simulink model "GaN_Full_Bridge_SPS"  (R2022b)
settings: Solver=ode45  StartTime=0.0  StopTime=55e-6  MaxStep=5e-9  RelTol=1e-7  AbsTol=1e-8
model workspace (MAT data in the model file):
  p.VDC = 150
  p.L = 9e-05
  p.Cdc = 0.0005
  p.Ron = 0.08
  p.Rdut = 0.08
  p.Raux = 0.08
  p.Rshunt = 0.01
  p.Rload = 0.001
  p.T0 = 2e-06
  p.Tcharge = 3.25e-05
  p.Tfree = 1e-06
  p.Tmeasure = 5e-06
  p.direction = 1
  p.conventional = 0
  p.idleUpper = 1
values from neighbouring files (symbols this model uses):
  p = h.(side)(index);end    [build_and_run_simulink.m]    (also in run_bridge_snapshot.m = evalin(w,'p'))
libraries: spsIdealSwitchLib x5, spsSeriesRLCBranchLib x3, spsVoltageMeasurementLib x2, spsCurrentMeasurementLib x2, spsGroundLib x1, sps_lib x1
settings Model: Creator=Greatlovers  LastModifiedBy=Greatlovers

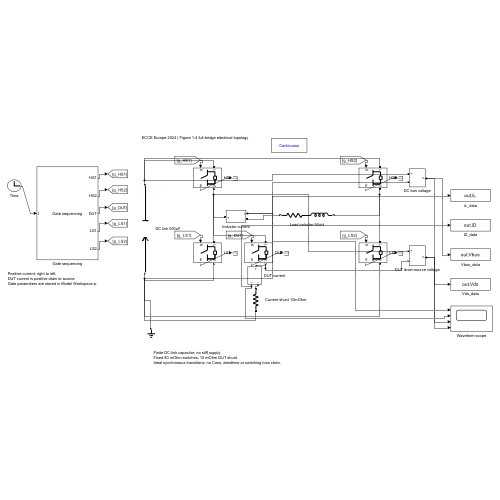
[thumbnail: Simulink's stored preview of the top-level diagram]
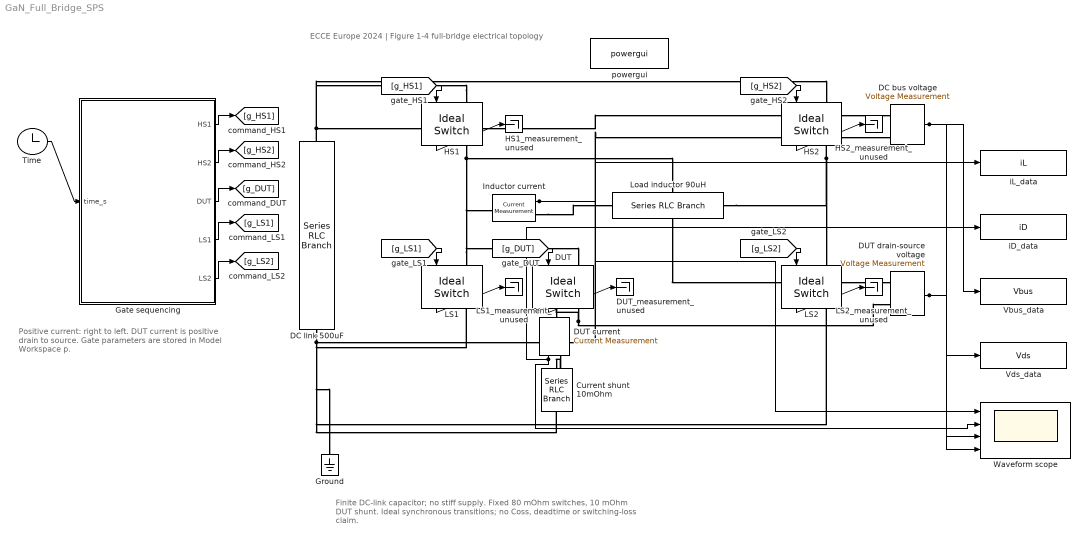
== system GaN_Full_Bridge_SPS ==
  note: ECCE Europe 2024 | Figure 1-4 full-bridge electrical topology
  note: Finite DC-link capacitor; no stiff supply.
      | Fixed 80 mOhm switches, 10 mOhm DUT shunt.
      | Ideal synchronous transitions; no Coss, deadtime or switching-loss claim.
  note: Positive current: right to left.
      | DUT current is positive drain to source.
      | Gate parameters are stored in Model Workspace p.
  Current shunt 10mOhm : spsSeriesRLCBranchLib/Series RLC Branch  LConnTagsString=__new0  RConnTagsString=__new0  BranchType=R  Resistance=p.Rshunt  Inductance=1e-3  SetiL0=off  InitialCurrent=0  Capacitance=1e-6  Setx0=off  InitialVoltage=0  Measurements=None
  DC bus voltage : spsVoltageMeasurementLib/Voltage Measurement  PhasorSimulation=off  OutputType=Complex  PSBequivalent=0
  DC link 500uF : spsSeriesRLCBranchLib/Series RLC Branch  LConnTagsString=__new0  RConnTagsString=__new0  BranchType=C  Resistance=1  Inductance=1e-3  SetiL0=off  InitialCurrent=0  Capacitance=p.Cdc  Setx0=on  InitialVoltage=p.VDC  Measurements=None
  DUT : spsIdealSwitchLib/Ideal Switch  Ron=p.Rdut  Lon=0  IC=0  Rs=1e9  Cs=inf  Measurements=on
  DUT current : spsCurrentMeasurementLib/Current Measurement  PhasorSimulation=off  OutputType=Complex  PSBequivalent=0
  DUT drain-source voltage : spsVoltageMeasurementLib/Voltage Measurement  PhasorSimulation=off  OutputType=Complex  PSBequivalent=0
  DUT_measurement_unused : Terminator
  Gate sequencing : Subsystem
      mask Display: disp('Gate sequencing');port_label('input',1,'t');port_label('output',1,'HS1');port_label('output',2,'HS2');port_label('output',3,'DUT');port_label('output',4,'LS1');port_label('output',5,'LS2');
  Ground : spsGroundLib/Ground  LConnTagsString=a
  HS1 : spsIdealSwitchLib/Ideal Switch  Ron=p.Raux  Lon=0  IC=0  Rs=1e9  Cs=inf  Measurements=on
  HS1_measurement_unused : Terminator
  HS2 : spsIdealSwitchLib/Ideal Switch  Ron=p.Raux  Lon=0  IC=0  Rs=1e9  Cs=inf  Measurements=on
  HS2_measurement_unused : Terminator
  Inductor current : spsCurrentMeasurementLib/Current Measurement  PhasorSimulation=off  OutputType=Complex  PSBequivalent=0
  LS1 : spsIdealSwitchLib/Ideal Switch  Ron=p.Raux  Lon=0  IC=0  Rs=1e9  Cs=inf  Measurements=on
  LS1_measurement_unused : Terminator
  LS2 : spsIdealSwitchLib/Ideal Switch  Ron=p.Raux  Lon=0  IC=0  Rs=1e9  Cs=inf  Measurements=on
  LS2_measurement_unused : Terminator
  Load inductor 90uH : spsSeriesRLCBranchLib/Series RLC Branch  LConnTagsString=__new0  RConnTagsString=__new0  BranchType=RL  Resistance=p.Rload  Inductance=p.L  SetiL0=on  InitialCurrent=0  Capacitance=1e-6  Setx0=off  InitialVoltage=0  Measurements=None
  Time : Clock
  Vbus_data : ToWorkspace  VariableName=Vbus  SaveFormat=Timeseries  SampleTime=-1
  Vds_data : ToWorkspace  VariableName=Vds  SaveFormat=Timeseries  SampleTime=-1
  Waveform scope : Scope  NumInputPorts=4
  iD_data : ToWorkspace  VariableName=iD  SaveFormat=Timeseries  SampleTime=-1
  iL_data : ToWorkspace  VariableName=iL  SaveFormat=Timeseries  SampleTime=-1
  powergui : sps_lib/powergui  Priority=1  SimulationMode=Continuous  SampleTime=50e-6  frequency=60  Iterations=50  frequencyindice=60  Pbase=100e6  ErrMax=1e-4  UnitsV=kV  UnitsW=MW  buscounter=0  FunctionMessages=off  echomessages=off  EnableUseOfTLC=off  CurrentSourceSwitches=off  DisableSnubberDevices=off  DisableRonSwitches=off  DisableVfSwitches=off  DisplayEquations=off  AutomaticDiscreteSolvers=off  SolverType=Tustin/Backward Euler (TBE)  Interpol=off  ExternalGateDelay=off  methode=off  Ts=100  x0status=blocks  SPID=on  SwTol=0  HookPort=off  NonlinearTolerance=1e-4  nMaxIteration=100  ContinueOnMaxIteration=off  RestoreLinks=warning  ResistiveCurrentMeasurement=off  Frange=[0:2:500]  Ylog=off  Xlog=on  ShowGrid=off  save=off  variable=ZData  structure=0  ZoomFFT=off  StartTime=0.0  cycles=1  DisplayStyle=1  fundamental=60  FreqAxis=off  MaxFrequency=1000  frequencyindicesteady=1  RmsSteady=1  display=off
  wires:
  Time/1 -> Gate sequencing/1(time_s)
  HS1/1 -> HS1_measurement_unused/1
  HS2/1 -> HS2_measurement_unused/1
  DUT/1 -> DUT_measurement_unused/1
  LS1/1 -> LS1_measurement_unused/1
  LS2/1 -> LS2_measurement_unused/1
  Inductor current/1 -> iL_data/1, Waveform scope/1
  DUT current/1 -> iD_data/1, Waveform scope/2
  DC bus voltage/1 -> Vbus_data/1, Waveform scope/3
  DUT drain-source voltage/1 -> Vds_data/1, Waveform scope/4
  Gate sequencing/1(HS1) -> [g_HS1]
  [g_HS1] -> HS1/1
  Gate sequencing/2(HS2) -> [g_HS2]
  [g_HS2] -> HS2/1
  Gate sequencing/3(DUT) -> [g_DUT]
  [g_DUT] -> DUT/1
  Gate sequencing/4(LS1) -> [g_LS1]
  [g_LS1] -> LS1/1
  Gate sequencing/5(LS2) -> [g_LS2]
  [g_LS2] -> LS2/1
  connections:
  HS1/LConn1 -- DC link 500uF/LConn1 -- HS2/LConn1 -- DC bus voltage/LConn1
  LS1/LConn1 -- HS1/RConn1 -- DUT/LConn1 -- Inductor current/LConn1 -- DUT drain-source voltage/LConn1
  Inductor current/RConn1 -- Load inductor 90uH/LConn1
  HS2/RConn1 -- Load inductor 90uH/RConn1 -- LS2/LConn1
  DUT current/LConn1 -- DUT/RConn1 -- DUT drain-source voltage/LConn2
  DUT current/RConn1 -- Current shunt 10mOhm/LConn1
  LS1/RConn1 -- DC link 500uF/RConn1 -- LS2/RConn1 -- Current shunt 10mOhm/RConn1 -- Ground/LConn1 -- DC bus voltage/LConn2

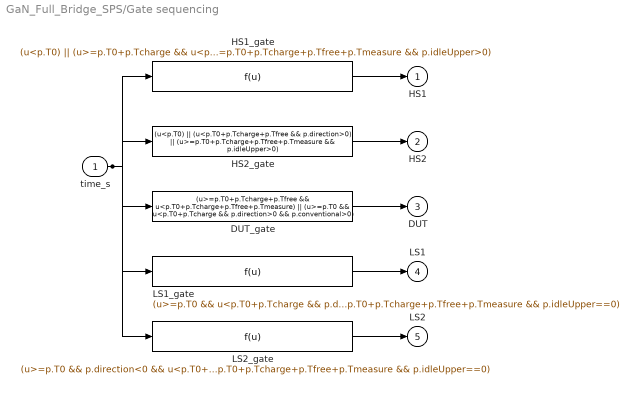
== system GaN_Full_Bridge_SPS/Gate sequencing ==
  time_s : Inport
  DUT_gate : Fcn  Expr=(u>=p.T0+p.Tcharge+p.Tfree && u<p.T0+p.Tcharge+p.Tfree+p.Tmeasure) || (u>=p.T0 && u<p.T0+p.Tcharge && p.direction>0 && p.conventional>0)
  HS1_gate : Fcn  Expr=(u<p.T0) || (u>=p.T0+p.Tcharge && u<p.T0+p.Tcharge+p.Tfree && p.direction>0) || (u>=p.T0 && u<p.T0+p.Tcharge && p.direction<0) || (u>=p.T0+p.Tcharge+p.Tfree+p.Tmeasure && p.idleUpper>0)
  HS2_gate : Fcn  Expr=(u<p.T0) || (u<p.T0+p.Tcharge+p.Tfree && p.direction>0) || (u>=p.T0+p.Tcharge+p.Tfree+p.Tmeasure && p.idleUpper>0)
  LS1_gate : Fcn  Expr=(u>=p.T0 && u<p.T0+p.Tcharge && p.direction>0 && p.conventional==0) || (u>=p.T0+p.Tcharge+p.Tfree+p.Tmeasure && p.idleUpper==0)
  LS2_gate : Fcn  Expr=(u>=p.T0 && p.direction<0 && u<p.T0+p.Tcharge+p.Tfree+p.Tmeasure) || (u>=p.T0+p.Tcharge+p.Tfree && u<p.T0+p.Tcharge+p.Tfree+p.Tmeasure) || (u>=p.T0+p.Tcharge+p.Tfree+p.Tmeasure && p.idleUpper==0)
  HS1 : Outport
  HS2 : Outport  Port=2
  DUT : Outport  Port=3
  LS1 : Outport  Port=4
  LS2 : Outport  Port=5
  wires:
  time_s/1 -> HS1_gate/1, HS2_gate/1, DUT_gate/1, LS1_gate/1, LS2_gate/1
  HS1_gate/1 -> HS1/1
  HS2_gate/1 -> HS2/1
  DUT_gate/1 -> DUT/1
  LS1_gate/1 -> LS1/1
  LS2_gate/1 -> LS2/1
